simulink model "sl_quadcopter_vs"  (Simulink 7.9)
settings: Solver=ode45  StartTime=0.0  StopTime=10.0  RelTol=1e-3
InitFcn:
  | fprintf('----- creating workspace variables: camera, quad, P, pstar\n');
  | % create a spherical camera
  | camera = SphericalCamera('name', 'quad-vs');
  | 
  | % create a grid of points on the ground
  | P = mkgrid(2, 4);
  | 
  | % set the desired view of these points, defines the final pose
  | % of the quad
  | pstar = camera.project(P, 'Tcam', transl(0, 0, -5)*trotz(pi/2));
  | 
  | % load a dynamic model of the quadcopter
  | mdl_quadcopter
undefined symbols (not defined in the file): rpy2tr, transl
libraries: roblocks x6
settings Model: Creator=corkep  LastModifiedBy=corkep
settings DebuggingCC: FcnCallInpInsideContextMsg=Use local settings
settings GRTTargetCC: CombineOutputUpdateFcns=off  GRTInterface=on

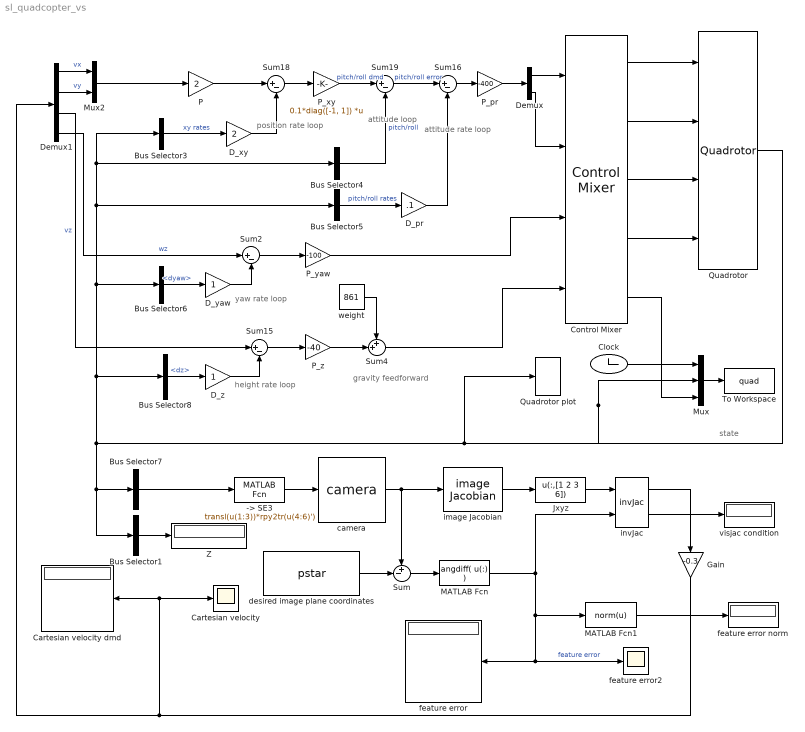
== system sl_quadcopter_vs ==
  note: state
  note: gravity feedforward
  note: attitude rate
      | loop
  note: attitude
      | loop
  note: position rate
      | loop
  note: yaw rate
      | loop
  note: height rate
      | loop
  -> SE3 : MATLABFcn  MATLABFcn=transl(u(1:3))*rpy2tr(u(4:6)')  OutputDimensions=[4 4]  Output1D=off
  Bus Selector1 : BusSelector  OutputSignals=Z  OutputAsBus=on
  Bus Selector3 : BusSelector  OutputSignals=dx,dy  OutputAsBus=on
  Bus Selector4 : BusSelector  OutputSignals=pitch,roll  OutputAsBus=on
  Bus Selector5 : BusSelector  OutputSignals=dpitch,droll  OutputAsBus=on
  Bus Selector6 : BusSelector  OutputSignals=dyaw
  Bus Selector7 : BusSelector  OutputSignals=X,Y,Z,roll,pitch,yaw  OutputAsBus=on
  Bus Selector8 : BusSelector  OutputSignals=dz
  Cartesian velocity : Scope
      settings: TimeRange=20  YMin=-0.4  YMax=1.9
  Cartesian velocity dmd : Display
      settings: Format=short_e
  Clock : Clock
  Control Mixer : roblocks/Dynamics/Control Mixer
  D_pr : Gain  Gain=.1
  D_xy : Gain  Gain=2
  D_yaw : Gain
  D_z : Gain
  Demux : Demux  Outputs=2
  Demux1 : Demux
  Gain : Gain  Gain=-0.3
  Jxyz : MATLABFcn  MATLABFcn=u(:,[1 2 3 6])  Output1D=off
  MATLAB Fcn : MATLABFcn  MATLABFcn=angdiff( u(:) )  Output1D=off
  MATLAB Fcn1 : MATLABFcn  MATLABFcn=norm(u)
  Mux : Mux  Inputs=3
  Mux2 : Mux  Inputs=2
  P : Gain  Gain=2
  P_pr : Gain  Gain=-400
  P_xy : Gain  Gain=0.1*diag([-1, 1])  Multiplication=Matrix(K*u)
  P_yaw : Gain  Gain=-100
  P_z : Gain  Gain=-40
  Quadrotor : roblocks/Dynamics/Quadrotor  quad=quad
  Quadrotor plot : roblocks/Robot Graphics/Quadrotor plot  x=0
  Sum : Sum  Inputs=+-|  SaturateOnIntegerOverflow=on  InputSameDT=on  OutDataTypeStr=Inherit: Same as first input
  Sum{2,15..16,18..19} (5 alike) : Sum  Inputs=|+-
  Sum4 : Sum  Inputs=++|
  To Workspace : ToWorkspace  VariableName=quad  SampleTime=-1
  Z : Display
  camera : roblocks/Vision/camera  cam=camera  points=P
  desired image plane coordinates : Constant  Value=pstar  VectorParams1D=off
  feature error : Display
      settings: Format=bank
  feature error norm : Display
  feature error2 : Scope
      settings: TimeRange=20  YMin=-150  YMax=150
  image Jacobian : roblocks/Vision/image Jacobian  cam=camera  z=2
  invJac : roblocks/Vision/invJac
  visjac condition : Display
  weight : Constant  Value=861  SampleTime=0
  wires:
  camera/1 -> Sum/1, image Jacobian/1
  Sum/1 -> MATLAB Fcn/1
  desired image plane coordinates/1 -> Sum/2
  MATLAB Fcn/1 -> MATLAB Fcn1/1, feature error2/1, feature error/1, invJac/2  "feature error"
  image Jacobian/1 -> Jxyz/1
  Jxyz/1 -> invJac/1
  -> SE3/1 -> camera/1
  Bus Selector7/1 -> -> SE3/1
  MATLAB Fcn1/1 -> feature error norm/1
  Demux1/1 -> Mux2/1  "vx"
  Demux1/2 -> Mux2/2  "vy"
  Gain/1 -> Cartesian velocity dmd/1, Cartesian velocity/1, Demux1/1
  Bus Selector1/1 -> Z/1
  Control Mixer/1 -> Quadrotor/1
  Control Mixer/3 -> Quadrotor/3
  Control Mixer/4 -> Quadrotor/4
  weight/1 -> Sum4/1
  Sum15/1 -> P_z/1
  P_z/1 -> Sum4/2
  Quadrotor/1 -> Bus Selector8/1, Bus Selector5/1, Bus Selector4/1, Bus Selector3/1, Bus Selector6/1, Bus Selector1/1, Bus Selector7/1, Quadrotor plot/1, Mux/2
  Bus Selector3/1 -> D_xy/1  "xy rates"
  D_xy/1 -> Sum18/2
  P_xy/1 -> Sum19/1  "pitch/roll dmd"
  Bus Selector4/1 -> Sum19/2  "pitch/roll"
  Bus Selector5/1 -> D_pr/1  "pitch/roll rates"
  Sum19/1 -> Sum16/1  "pitch/roll error"
  Sum16/1 -> P_pr/1
  P_pr/1 -> Demux/1
  P_yaw/1 -> Control Mixer/3
  Sum2/1 -> P_yaw/1
  Bus Selector6/1 -> D_yaw/1  "<dyaw>"
  Bus Selector8/1 -> D_z/1  "<dz>"
  D_z/1 -> Sum15/2
  D_pr/1 -> Sum16/2
  Demux/2 -> Control Mixer/2
  Demux/1 -> Control Mixer/1
  D_yaw/1 -> Sum2/2
  Sum4/1 -> Control Mixer/4
  Control Mixer/2 -> Quadrotor/2
  Mux/1 -> To Workspace/1
  Clock/1 -> Mux/1
  Control Mixer/5 -> Mux/3
  Sum18/1 -> P_xy/1
  Mux2/1 -> P/1
  Demux1/3 -> Sum15/1  "vz"
  Demux1/4 -> Sum2/1  "wz"
  invJac/1 -> Gain/1
  invJac/2 -> visjac condition/1
  P/1 -> Sum18/1
